simulink model "Simulator_Single_Axis"  (R2025b)
settings: Solver=FixedStepAuto  StartTime=0.0  StopTime=simulation_time  RelTol=1e-6  AbsTol=1e-6
values from neighbouring files (symbols this model uses):
  A = [Xu, Xq, -9.81; Mu, Mq, 0; 0, 1, 0]    [main_quad_ANTX.m]
  B = [Xd; Md; 0]    [main_quad_ANTX.m]
  BASELINE_T = 0.4    [parameters_controller.m]
  C = [1, 0, 0; 0, 1, 0; 0, 0, 1; Xu, Xq, 0]    [main_quad_ANTX.m]
  D = [0; 0; 0; Xd]    [main_quad_ANTX.m]
  KD_Q = 0.0016    [parameters_controller.m]
  KD_X_DOT = 0    [parameters_controller.m]
  KI_Q = 0.21    [parameters_controller.m]
  KI_X_DOT = 0.04    [parameters_controller.m]
  KP_PITCH = 12    [parameters_controller.m]
  KP_Q = 0.09    [parameters_controller.m]
  KP_X = 2    [parameters_controller.m]
  KP_X_DOT = 0.5    [parameters_controller.m]
  N_filter_rate = 100    [parameters_controller.m]
  N_filter_vel = 10    [parameters_controller.m]
  Q_MAX = 10    [parameters_controller.m]
  Q_MIN = -10    [parameters_controller.m]
  sample_time = 1/250    (= 0.004)    [parameters_controller.m]
  VEL_MAX = 10    [parameters_controller.m]
  VEL_MIN = -10    [parameters_controller.m]
undefined symbols (not defined in the file or in its folder): delay, noise, sim_seed
libraries: custom_PIDs_w_reset x4
settings Model: Creator=SalvatoreMeraglia  LastModifiedBy=mghor
settings SolverCC: AlgebraicLoopSolver=TrustRegion
settings DebuggingCC: UnconnectedInputMsg=warning  UnconnectedOutputMsg=warning  UnconnectedLineMsg=warning
settings ModelReferenceCC: EnableRefExpFcnMdlSchedulingChecks=on
settings RTWCC: GPUComputeCapability=3.5  DLArmComputeVersion=19.05

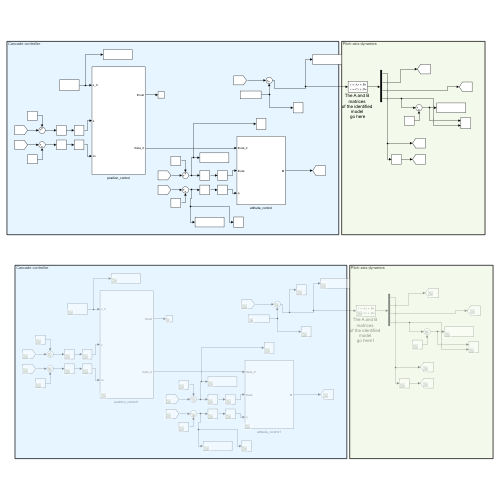
[thumbnail: Simulink's stored preview of the top-level diagram]
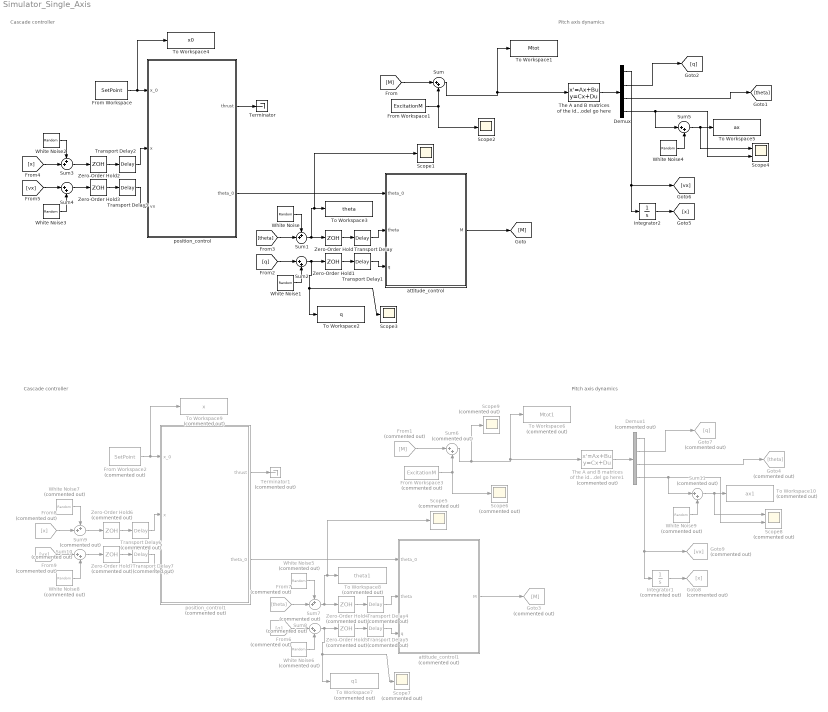
== system Simulator_Single_Axis ==
  note: Cascade controller
  note: Pitch axis dynamics
  note: Cascade controller
  note: Pitch axis dynamics
  Demux : Demux
  Demux1 : Demux  Commented=on
  From Workspace : FromWorkspace  VariableName=SetPoint  SampleTime=sample_time  OutputAfterFinalValue=Setting to zero
  From Workspace1 : FromWorkspace  VariableName=ExcitationM  SampleTime=sample_time  OutputAfterFinalValue=Setting to zero
  From Workspace2 : FromWorkspace  Commented=on  VariableName=SetPoint  SampleTime=sample_time  OutputAfterFinalValue=Setting to zero
  From Workspace3 : FromWorkspace  Commented=on  VariableName=ExcitationM  SampleTime=sample_time  OutputAfterFinalValue=Setting to zero
  From1 : From  Commented=on  GotoTag=M
  From6 : From  Commented=on  GotoTag=q
  From7 : From  Commented=on  GotoTag=theta
  From8 : From  Commented=on  GotoTag=x
  From9 : From  Commented=on  GotoTag=vx
  Goto3 : Goto  Commented=on  GotoTag=M
  Goto4 : Goto  Commented=on  GotoTag=theta
  Goto7 : Goto  Commented=on  GotoTag=q
  Goto8 : Goto  Commented=on  GotoTag=x
  Goto9 : Goto  Commented=on  GotoTag=vx
  Integrator1 : Integrator  Commented=on
  Integrator2 : Integrator
  Scope1 : Scope
      settings: ActiveDisplayYMinimum=-2.36747  ActiveDisplayYMaximum=2.35714
  Scope2 : Scope
      settings: ActiveDisplayYMinimum=-1  ActiveDisplayYMaximum=1
  Scope3 : Scope
      settings: ActiveDisplayYMinimum=-14.48365  ActiveDisplayYMaximum=14.03518
  Scope4 : Scope  NumInputPorts=2
      settings: ActiveDisplayYMinimum=-2.36747  ActiveDisplayYMaximum=2.35714
  Scope{5..7,9} (4 alike) : Scope  Commented=on
      Scope5 settings: ActiveDisplayYMinimum=-2.36747  ActiveDisplayYMaximum=2.35714  DataLoggingVariableName=ScopeData2
      Scope6 settings: ActiveDisplayYMinimum=-1  ActiveDisplayYMaximum=1  DataLoggingVariableName=ScopeData3
      Scope7 settings: ActiveDisplayYMinimum=-14.48365  ActiveDisplayYMaximum=14.03518  DataLoggingVariableName=ScopeData4
      Scope9 settings: ActiveDisplayYMinimum=-0.12157812741241911  ActiveDisplayYMaximum=0.12307917245953474
  Scope8 : Scope  Commented=on  NumInputPorts=2
      settings: ActiveDisplayYMinimum=-2.36747  ActiveDisplayYMaximum=2.35714  DataLoggingVariableName=ScopeData5
  Sum{,2,4..5} (4 alike) : Sum  Inputs=|++
  Sum1 : Sum  Inputs=++|
  Sum{6,8,10..11} (4 alike) : Sum  Commented=on  Inputs=|++
  Sum3 : Sum  Inputs=++|
  Sum7 : Sum  Commented=on  Inputs=++|
  Sum9 : Sum  Commented=on  Inputs=++|
  Terminator : Terminator
  Terminator1 : Terminator  Commented=on
  The A and B matrices of the identified model go here : StateSpace  A=A  B=B  C=C  D=D  InitialCondition=0
  The A and B matrices of the identified model go here1 : StateSpace  Commented=on  A=A  B=B  C=C  D=D  InitialCondition=0
  To Workspace1 : ToWorkspace  VariableName=Mtot  SaveFormat=Timeseries  SampleTime=sample_time
  To Workspace10 : ToWorkspace  Commented=on  VariableName=ax1  SaveFormat=Timeseries  SampleTime=sample_time
  To Workspace2 : ToWorkspace  VariableName=q  SaveFormat=Timeseries  SampleTime=sample_time
  To Workspace3 : ToWorkspace  VariableName=theta  SampleTime=sample_time
  To Workspace4 : ToWorkspace  VariableName=x0  SampleTime=sample_time
  To Workspace5 : ToWorkspace  VariableName=ax  SaveFormat=Timeseries  SampleTime=sample_time
  To Workspace6 : ToWorkspace  Commented=on  VariableName=Mtot1  SaveFormat=Timeseries  SampleTime=sample_time
  To Workspace7 : ToWorkspace  Commented=on  VariableName=q1  SaveFormat=Timeseries  SampleTime=sample_time
  To Workspace8 : ToWorkspace  Commented=on  VariableName=theta1  SampleTime=sample_time
  To Workspace9 : ToWorkspace  Commented=on  VariableName=x  SampleTime=sample_time
  Transport Delay : TransportDelay  DelayTime=delay.attitude_filter * sample_time
  Transport Delay1 : TransportDelay  DelayTime=delay.attitude_filter * sample_time
  Transport Delay2 : TransportDelay  DelayTime=delay.position_filter * sample_time
  Transport Delay3 : TransportDelay  DelayTime=delay.position_filter * sample_time
  Transport Delay4 : TransportDelay  Commented=on  DelayTime=delay.attitude_filter * sample_time
  Transport Delay5 : TransportDelay  Commented=on  DelayTime=delay.attitude_filter * sample_time
  Transport Delay6 : TransportDelay  Commented=on  DelayTime=delay.position_filter * sample_time
  Transport Delay7 : TransportDelay  Commented=on  DelayTime=delay.position_filter * sample_time
  White Noise : RandomNumber  DisableCoverage=on  Variance=noise.attitude_stand_dev^2  Seed=sim_seed + 1  SampleTime=sample_time
  White Noise1 : RandomNumber  DisableCoverage=on  Variance=noise.ang_rate_stand_dev^2  Seed=sim_seed + 2  SampleTime=sample_time
  White Noise2 : RandomNumber  DisableCoverage=on  Variance=noise.pos_stand_dev^2  Seed=sim_seed + 3  SampleTime=sample_time
  White Noise3 : RandomNumber  DisableCoverage=on  Variance=noise.vel_stand_dev^2  Seed=sim_seed + 4  SampleTime=sample_time
  White Noise4 : RandomNumber  DisableCoverage=on  Variance=noise.acc_stand_dev^2  Seed=sim_seed + 5  SampleTime=sample_time
  White Noise5 : RandomNumber  Commented=on  DisableCoverage=on  Variance=noise.attitude_stand_dev^2  Seed=sim_seed  SampleTime=sample_time
  White Noise6 : RandomNumber  Commented=on  DisableCoverage=on  Variance=noise.ang_rate_stand_dev^2  Seed=sim_seed  SampleTime=sample_time
  White Noise7 : RandomNumber  Commented=on  DisableCoverage=on  Variance=noise.pos_stand_dev^2  Seed=sim_seed  SampleTime=sample_time
  White Noise8 : RandomNumber  Commented=on  DisableCoverage=on  Variance=noise.vel_stand_dev^2  Seed=sim_seed  SampleTime=sample_time
  White Noise9 : RandomNumber  Commented=on  DisableCoverage=on  Variance=noise.acc_stand_dev^2  Seed=sim_seed  SampleTime=sample_time
  Zero-Order Hold{,1..3} (4 alike) : ZeroOrderHold  SampleTime=sample_time
  Zero-Order Hold{4..7} (4 alike) : ZeroOrderHold  Commented=on  SampleTime=sample_time
  attitude_control : Subsystem
  attitude_control1 : Subsystem  Commented=on
  position_control : Subsystem
  position_control1 : Subsystem  Commented=on
  wires:
  Transport Delay2/1 -> position_control/2(x)
  Transport Delay3/1 -> position_control/3(vx)
  attitude_control/1(M) -> [M]
  position_control/2(theta_0) -> attitude_control/1(theta_0)
  position_control/1(thrust) -> Terminator/1
  Demux/3 -> [theta]
  [M] -> Sum/1
  Sum/1 -> The A and B matrices of the identified model go here/1, To Workspace1/1
  From Workspace/1 -> To Workspace4/1, position_control/1(x_0)
  From Workspace1/1 -> Scope2/1, Sum/2
  Zero-Order Hold1/1 -> Transport Delay1/1
  White Noise2/1 -> Sum3/1
  [theta] -> Sum1/2
  White Noise/1 -> Sum1/1
  Zero-Order Hold/1 -> Transport Delay/1
  [vx] -> Sum4/1
  White Noise3/1 -> Sum4/2
  Sum3/1 -> Zero-Order Hold2/1
  [x] -> Sum3/2
  Zero-Order Hold2/1 -> Transport Delay2/1
  Sum2/1 -> Scope3/1, To Workspace2/1, Zero-Order Hold1/1
  [q] -> Sum2/1
  Zero-Order Hold3/1 -> Transport Delay3/1
  Sum4/1 -> Zero-Order Hold3/1
  Sum1/1 -> Scope1/1, To Workspace3/1, Zero-Order Hold/1
  White Noise1/1 -> Sum2/2
  Transport Delay1/1 -> attitude_control/3(q)
  Transport Delay/1 -> attitude_control/2(theta)
  The A and B matrices of the identified model go here/1 -> Demux/1
  Demux/2 -> [q]
  Demux/1 -> [vx], Integrator2/1
  Integrator2/1 -> [x]
  White Noise4/1 -> Sum5/2
  Sum5/1 -> Scope4/1, To Workspace5/1
  Demux/4 -> Scope4/2, Sum5/1
  Sum6/1 -> Scope9/1, The A and B matrices of the identified model go here1/1, To Workspace6/1
  Demux1/4 -> Scope8/2, Sum11/1
  Sum9/1 -> Zero-Order Hold6/1
  Sum10/1 -> Zero-Order Hold7/1
  From9/1 -> Sum10/1
  Transport Delay4/1 -> attitude_control1/2(theta)
  From Workspace2/1 -> To Workspace9/1, position_control1/1(x_0)
  Demux1/1 -> Goto9/1, Integrator1/1
  White Noise8/1 -> Sum10/2
  White Noise9/1 -> Sum11/2
  White Noise5/1 -> Sum7/1
  Sum11/1 -> Scope8/1, To Workspace10/1
  Zero-Order Hold4/1 -> Transport Delay4/1
  Zero-Order Hold5/1 -> Transport Delay5/1
  From Workspace3/1 -> Scope6/1, Sum6/2
  Demux1/3 -> Goto4/1
  Sum8/1 -> Scope7/1, To Workspace7/1, Zero-Order Hold5/1
  attitude_control1/1(M) -> Goto3/1
  White Noise7/1 -> Sum9/1
  Sum7/1 -> Scope5/1, To Workspace8/1, Zero-Order Hold4/1
  Zero-Order Hold6/1 -> Transport Delay6/1
  Demux1/2 -> Goto7/1
  The A and B matrices of the identified model go here1/1 -> Demux1/1
  Zero-Order Hold7/1 -> Transport Delay7/1
  From1/1 -> Sum6/1
  From8/1 -> Sum9/2
  From7/1 -> Sum7/2
  position_control1/2(theta_0) -> attitude_control1/1(theta_0)
  Transport Delay5/1 -> attitude_control1/3(q)
  Integrator1/1 -> Goto8/1
  Transport Delay6/1 -> position_control1/2(x)
  position_control1/1(thrust) -> Terminator1/1
  White Noise6/1 -> Sum8/2
  Transport Delay7/1 -> position_control1/3(vx)
  From6/1 -> Sum8/1

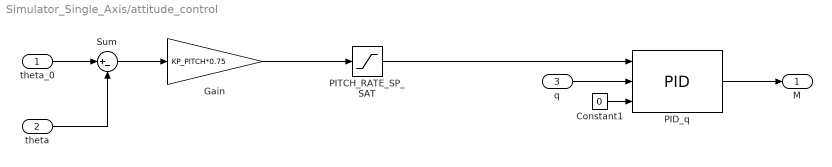
== system Simulator_Single_Axis/attitude_control ==
  theta_0 : Inport
  theta : Inport  Port=2
  q : Inport  Port=3
  Constant1 : Constant  Value=0  OutDataTypeStr=boolean
  Gain : Gain  Gain=KP_PITCH*0.75
  PID_q : custom_PIDs_w_reset/PID  Kf=KF_Q  Kp=KP_Q  Ki=KI_Q  Kd=KD_Q  N=N_filter_rate  min_u=M_MIN  max_u=M_MAX  ts=sample_time
  PITCH_RATE_SP_SAT : Saturate  UpperLimit=Q_MAX  LowerLimit=Q_MIN
  Sum : Sum  Inputs=|+-
  M : Outport
  wires:
  PID_q/1 -> M/1
  q/1 -> PID_q/2
  PITCH_RATE_SP_SAT/1 -> PID_q/1
  Sum/1 -> Gain/1
  theta_0/1 -> Sum/1
  theta/1 -> Sum/2
  Gain/1 -> PITCH_RATE_SP_SAT/1
  Constant1/1 -> PID_q/3

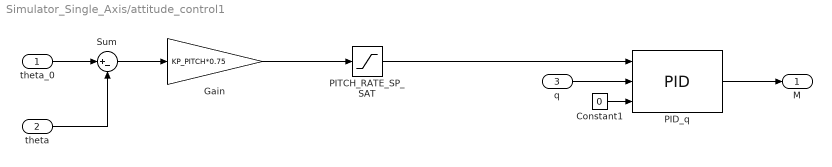
== system Simulator_Single_Axis/attitude_control1 ==
  theta_0 : Inport
  theta : Inport  Port=2
  q : Inport  Port=3
  Constant1 : Constant  Value=0  OutDataTypeStr=boolean
  Gain : Gain  Gain=KP_PITCH*0.75
  PID_q : custom_PIDs_w_reset/PID  Kf=KF_Q  Kp=KP_Q  Ki=KI_Q  Kd=KD_Q  N=N_filter_rate  min_u=M_MIN  max_u=M_MAX  ts=sample_time
  PITCH_RATE_SP_SAT : Saturate  UpperLimit=Q_MAX  LowerLimit=Q_MIN
  Sum : Sum  Inputs=|+-
  M : Outport
  wires:
  PID_q/1 -> M/1
  q/1 -> PID_q/2
  PITCH_RATE_SP_SAT/1 -> PID_q/1
  Sum/1 -> Gain/1
  theta_0/1 -> Sum/1
  theta/1 -> Sum/2
  Gain/1 -> PITCH_RATE_SP_SAT/1
  Constant1/1 -> PID_q/3

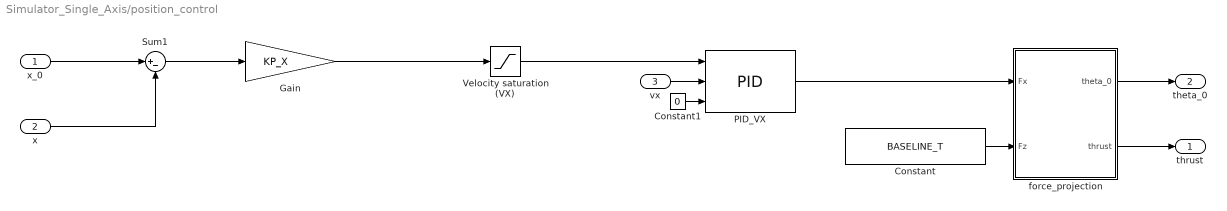
== system Simulator_Single_Axis/position_control ==
  x_0 : Inport
  x : Inport  Port=2
  vx : Inport  Port=3
  Constant : Constant  Value=BASELINE_T
  Constant1 : Constant  Value=0  OutDataTypeStr=boolean
  Gain : Gain  Gain=KP_X
  PID_VX : custom_PIDs_w_reset/PID  Kf=KF_X_DOT  Kp=KP_X_DOT  Ki=KI_X_DOT  Kd=KD_X_DOT  N=N_filter_vel  min_u=F_X_MIN  max_u=F_X_MAX  ts=sample_time
  Sum1 : Sum  Inputs=|+-
  Velocity saturation (VX) : Saturate  UpperLimit=VEL_MAX  LowerLimit=VEL_MIN
  force_projection : Subsystem
  thrust : Outport
  theta_0 : Outport  Port=2
  wires:
  vx/1 -> PID_VX/2
  Velocity saturation (VX)/1 -> PID_VX/1
  Sum1/1 -> Gain/1
  x_0/1 -> Sum1/1
  x/1 -> Sum1/2
  force_projection/2(thrust) -> thrust/1
  Gain/1 -> Velocity saturation (VX)/1
  Constant1/1 -> PID_VX/3
  Constant/1 -> force_projection/2(Fz)
  PID_VX/1 -> force_projection/1(Fx)
  force_projection/1(theta_0) -> theta_0/1

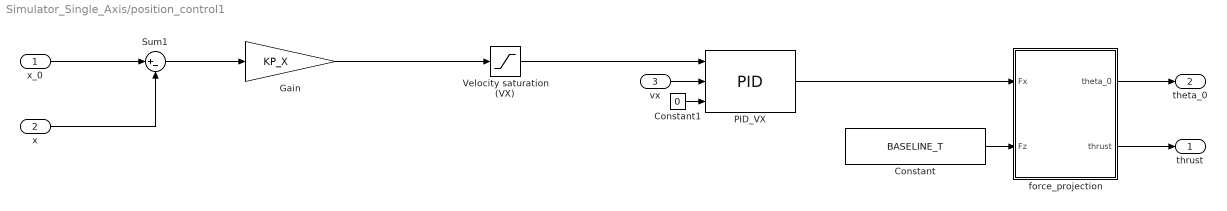
== system Simulator_Single_Axis/position_control1 ==
  x_0 : Inport
  x : Inport  Port=2
  vx : Inport  Port=3
  Constant : Constant  Value=BASELINE_T
  Constant1 : Constant  Value=0  OutDataTypeStr=boolean
  Gain : Gain  Gain=KP_X
  PID_VX : custom_PIDs_w_reset/PID  Kf=KF_X_DOT  Kp=KP_X_DOT  Ki=KI_X_DOT  Kd=KD_X_DOT  N=N_filter_vel  min_u=F_X_MIN  max_u=F_X_MAX  ts=sample_time
  Sum1 : Sum  Inputs=|+-
  Velocity saturation (VX) : Saturate  UpperLimit=VEL_MAX  LowerLimit=VEL_MIN
  force_projection : Subsystem
  thrust : Outport
  theta_0 : Outport  Port=2
  wires:
  vx/1 -> PID_VX/2
  Velocity saturation (VX)/1 -> PID_VX/1
  Sum1/1 -> Gain/1
  x_0/1 -> Sum1/1
  x/1 -> Sum1/2
  force_projection/2(thrust) -> thrust/1
  Gain/1 -> Velocity saturation (VX)/1
  Constant1/1 -> PID_VX/3
  Constant/1 -> force_projection/2(Fz)
  PID_VX/1 -> force_projection/1(Fx)
  force_projection/1(theta_0) -> theta_0/1

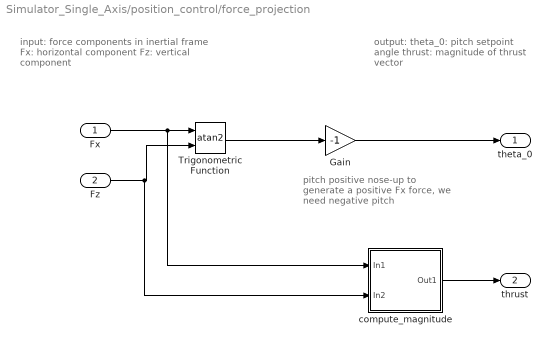
== system Simulator_Single_Axis/position_control/force_projection ==
  note: pitch positive nose-up
      | to generate a positive Fx force,
      | we need negative pitch
  note: output:
      | theta_0: pitch setpoint angle
      | thrust: magnitude of thrust vector
  note: input: force components in inertial frame
      | Fx: horizontal component
      | Fz: vertical component
  Fx : Inport
  Fz : Inport  Port=2
  Gain : Gain  Gain=-1
  Trigonometric Function : Trigonometry  Operator=atan2
  compute_magnitude : Subsystem
  theta_0 : Outport
  thrust : Outport  Port=2
  wires:
  Fx/1 -> compute_magnitude/1(In1), Trigonometric Function/1
  Fz/1 -> compute_magnitude/2(In2), Trigonometric Function/2
  Trigonometric Function/1 -> Gain/1
  Gain/1 -> theta_0/1
  compute_magnitude/1(Out1) -> thrust/1

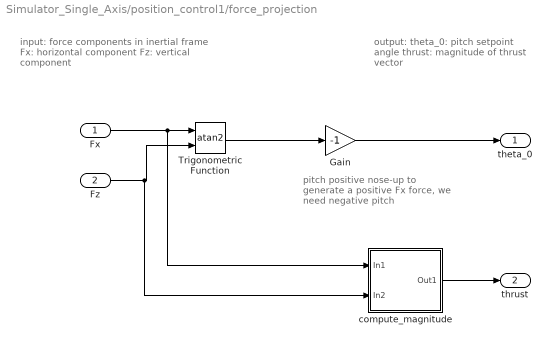
== system Simulator_Single_Axis/position_control1/force_projection ==
  note: pitch positive nose-up
      | to generate a positive Fx force,
      | we need negative pitch
  note: output:
      | theta_0: pitch setpoint angle
      | thrust: magnitude of thrust vector
  note: input: force components in inertial frame
      | Fx: horizontal component
      | Fz: vertical component
  Fx : Inport
  Fz : Inport  Port=2
  Gain : Gain  Gain=-1
  Trigonometric Function : Trigonometry  Operator=atan2
  compute_magnitude : Subsystem
  theta_0 : Outport
  thrust : Outport  Port=2
  wires:
  Fx/1 -> compute_magnitude/1(In1), Trigonometric Function/1
  Fz/1 -> compute_magnitude/2(In2), Trigonometric Function/2
  Trigonometric Function/1 -> Gain/1
  Gain/1 -> theta_0/1
  compute_magnitude/1(Out1) -> thrust/1

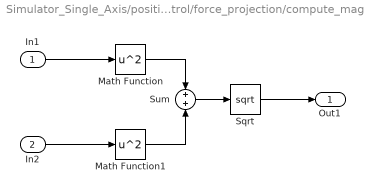
== system Simulator_Single_Axis/position_control/force_projection/compute_magnitude ==
  In1 : Inport
  In2 : Inport  Port=2
  Math Function : Math  Operator=square  SignedPower=on
  Math Function1 : Math  Operator=square  SignedPower=on
  Sqrt : Sqrt
  Sum : Sum
  Out1 : Outport
  wires:
  Sum/1 -> Sqrt/1
  Sqrt/1 -> Out1/1
  In1/1 -> Math Function/1
  Math Function1/1 -> Sum/2
  Math Function/1 -> Sum/1
  In2/1 -> Math Function1/1

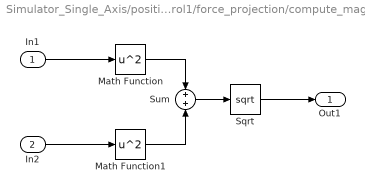
== system Simulator_Single_Axis/position_control1/force_projection/compute_magnitude ==
  In1 : Inport
  In2 : Inport  Port=2
  Math Function : Math  Operator=square  SignedPower=on
  Math Function1 : Math  Operator=square  SignedPower=on
  Sqrt : Sqrt
  Sum : Sum
  Out1 : Outport
  wires:
  Sum/1 -> Sqrt/1
  Sqrt/1 -> Out1/1
  In1/1 -> Math Function/1
  Math Function1/1 -> Sum/2
  Math Function/1 -> Sum/1
  In2/1 -> Math Function1/1
